simulink model "demo_package_drop"  (R2026a)
settings: Solver=FixedStepDiscrete  StopTime=2  FixedStep=.1
settings Model: Creator=harry_31916  LastModifiedBy=harry_31916

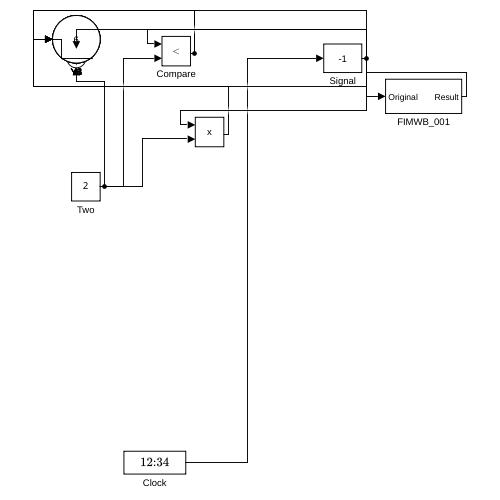
[thumbnail: Simulink's stored preview of the top-level diagram]
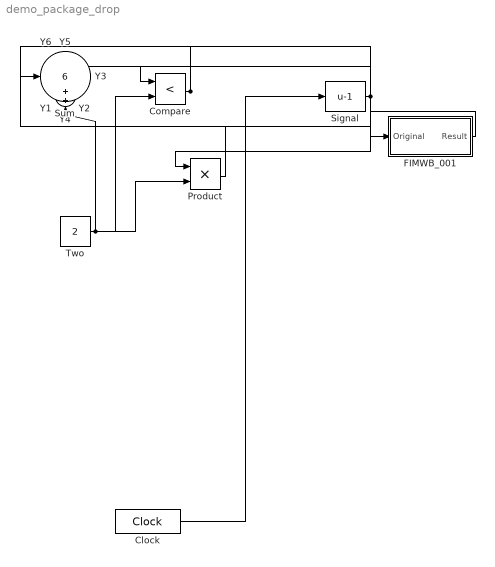
== system demo_package_drop ==
  Clock : DigitalClock  SampleTime=.1
  Compare : RelationalOperator  Operator=<  OutDataTypeStr=boolean  RndMeth=Simplest  InputSameDT=off
  FIMWB_001 : Subsystem  Tag=fimwb.fault.1
  Product : Product  Inputs=**
  Signal : Bias  Bias=-1  SaturateOnIntegerOverflow=off
  Sum : Sum
  Two : Constant  Value=2
  Y1 : Outport  SampleTime=0.1
  Y2 : Outport  Port=2  SampleTime=0.1
  Y3 : Outport  Port=3  SampleTime=0.1
  Y4 : Outport  Port=4  SampleTime=0.1
  Y5 : Outport  Port=5  SampleTime=0.1
  Y6 : Outport  Port=6  SampleTime=0.1
  wires:
  Clock/1 -> Signal/1
  Signal/1 -> Sum/1, Product/1, Compare/1, Y2/1, FIMWB_001/1(Original)
  Two/1 -> Sum/2, Product/2, Compare/2
  Sum/1 -> Y3/1
  Product/1 -> Y4/1
  Compare/1 -> Y5/1, Y6/1
  FIMWB_001/1(Result) -> Y1/1

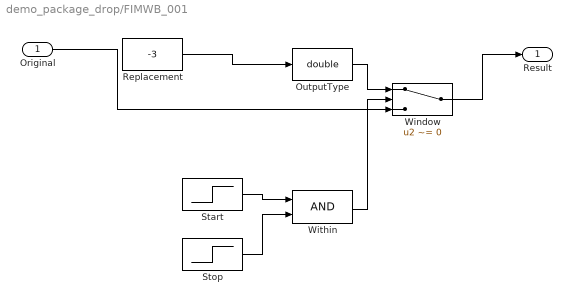
== system demo_package_drop/FIMWB_001 ==
  Original : Inport
  OutputType : DataTypeConversion  OutDataTypeStr=double  RndMeth=Round
  Replacement : Constant  Value=-3  OutDataTypeStr=double  SampleTime=[0.10000000000000001 0]
  Start : Step  Time=0.40000000000000002  SampleTime=0
  Stop : Step  InitialValue=1  FinalValue=0  SampleTime=0
  Window : Switch  Criteria=u2 ~= 0  SaturateOnIntegerOverflow=off  InputSameDT=off
  Within : Logic  AllPortsSameDT=off  OutDataTypeStr=boolean
  Result : Outport
  wires:
  Replacement/1 -> OutputType/1
  Start/1 -> Within/1
  Stop/1 -> Within/2
  OutputType/1 -> Window/1
  Within/1 -> Window/2
  Original/1 -> Window/3
  Window/1 -> Result/1
